simulink model "acc_sil"  (R2024b)
settings: Solver=ode4  StartTime=0.0  StopTime=T_sim  FixedStep=Ts  RelTol=1e-3
values from neighbouring files (symbols this model uses):
  Af = 2.2    [acc_params.m]    (also in build_acc_plant.m)
  Cd = 0.30    (= 0.3)    [acc_params.m]    (also in build_acc_plant.m)
  Crr = 0.012    [acc_params.m]    (also in build_acc_plant.m)
  g = 9.81    [acc_params.m]    (also in build_acc_plant.m)
  m = 1500    [acc_params.m]    (also in build_acc_plant.m)
  rho = 1.225    [acc_params.m]    (also in build_acc_plant.m)
  tau_pt = 0.30    (= 0.3)    [acc_params.m]    (also in build_acc_plant.m)
undefined symbols (not defined in the file or in its folder): sgn, v0_ego, x0_lead
settings Model: Creator=Aymen  LastModifiedBy=Aymen

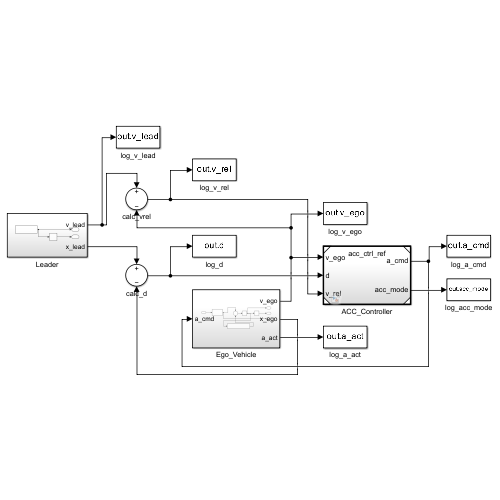
[thumbnail: Simulink's stored preview of the top-level diagram]
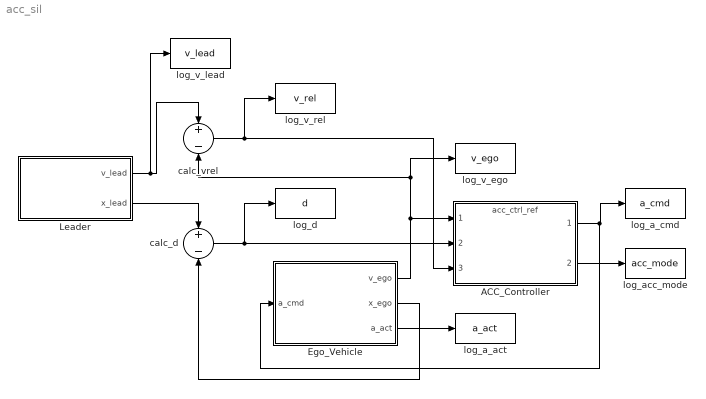
== system acc_sil ==
  ACC_Controller : ModelReference  ModelNameDialog=acc_ctrl_ref  SimulationMode=Normal  ModelReferenceVersion=1.7
  Ego_Vehicle : Subsystem
  Leader : Subsystem
  calc_d : Sum  Inputs=+-
  calc_vrel : Sum  Inputs=+-
  log_a_act : ToWorkspace  VariableName=a_act  SaveFormat=Timeseries  SampleTime=-1
  log_a_cmd : ToWorkspace  VariableName=a_cmd  SaveFormat=Timeseries  SampleTime=-1
  log_acc_mode : ToWorkspace  VariableName=acc_mode  SaveFormat=Timeseries  SampleTime=-1
  log_d : ToWorkspace  VariableName=d  SaveFormat=Timeseries  SampleTime=-1
  log_v_ego : ToWorkspace  VariableName=v_ego  SaveFormat=Timeseries  SampleTime=-1
  log_v_lead : ToWorkspace  VariableName=v_lead  SaveFormat=Timeseries  SampleTime=-1
  log_v_rel : ToWorkspace  VariableName=v_rel  SaveFormat=Timeseries  SampleTime=-1
  wires:
  Leader/2(x_lead) -> calc_d/1
  Leader/1(v_lead) -> calc_vrel/1, log_v_lead/1
  calc_vrel/1 -> ACC_Controller/3, log_v_rel/1
  Ego_Vehicle/2(x_ego) -> calc_d/2
  calc_d/1 -> ACC_Controller/2, log_d/1
  Ego_Vehicle/1(v_ego) -> calc_vrel/2, log_v_ego/1, ACC_Controller/1
  Ego_Vehicle/3(a_act) -> log_a_act/1
  ACC_Controller/1 -> Ego_Vehicle/1(a_cmd), log_a_cmd/1
  ACC_Controller/2 -> log_acc_mode/1

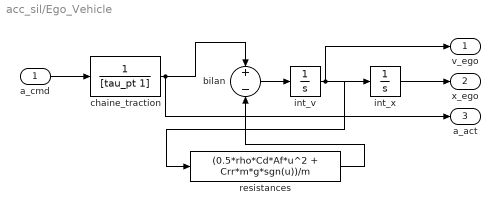
== system acc_sil/Ego_Vehicle ==
  a_cmd : Inport
  bilan : Sum  Inputs=+-
  chaine_traction : TransferFcn  Numerator=1  Denominator=[tau_pt 1]
  int_v : Integrator  InitialCondition=v0_ego  LimitOutput=on  LowerSaturationLimit=0
  int_x : Integrator
  resistances : Fcn  Expr=(0.5*rho*Cd*Af*u^2 + Crr*m*g*sgn(u))/m
  v_ego : Outport
  x_ego : Outport  Port=2
  a_act : Outport  Port=3
  wires:
  a_cmd/1 -> chaine_traction/1
  chaine_traction/1 -> bilan/1, a_act/1
  resistances/1 -> bilan/2
  bilan/1 -> int_v/1
  int_v/1 -> resistances/1, int_x/1, v_ego/1
  int_x/1 -> x_ego/1

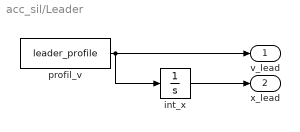
== system acc_sil/Leader ==
  int_x : Integrator  InitialCondition=x0_lead
  profil_v : FromWorkspace  VariableName=leader_profile  OutputAfterFinalValue=Holding final value
  v_lead : Outport
  x_lead : Outport  Port=2
  wires:
  profil_v/1 -> v_lead/1, int_x/1
  int_x/1 -> x_lead/1
